simulink subsystem "Swerve_Drive_Module_sub"  (R2023b)
settings: Solver=VariableStepAuto  StartTime=0.0  StopTime=10.0  RelTol=1e-3
undefined symbols (not defined in the file): Drive_Motor_Control_Module_Angle_Error, Drive_Motor_Control_Scale_Factor, Drive_Motor_Control_Sign_Change_Deadband, Wheel_Speed_to_Motor_Speed
libraries: Controls_Components_lib x4, simulink x2
settings Model: Creator=ander  LastModifiedBy=ander

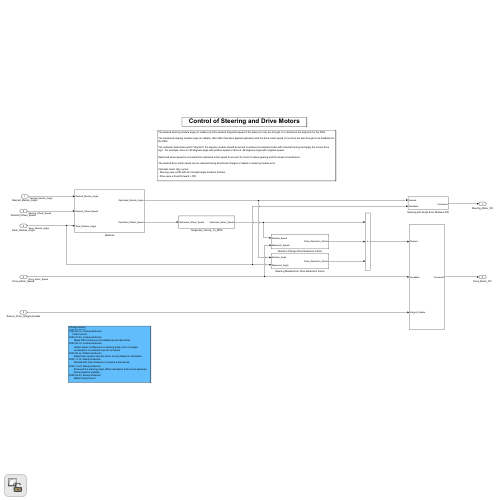
[thumbnail: Simulink's stored preview of the top-level diagram]
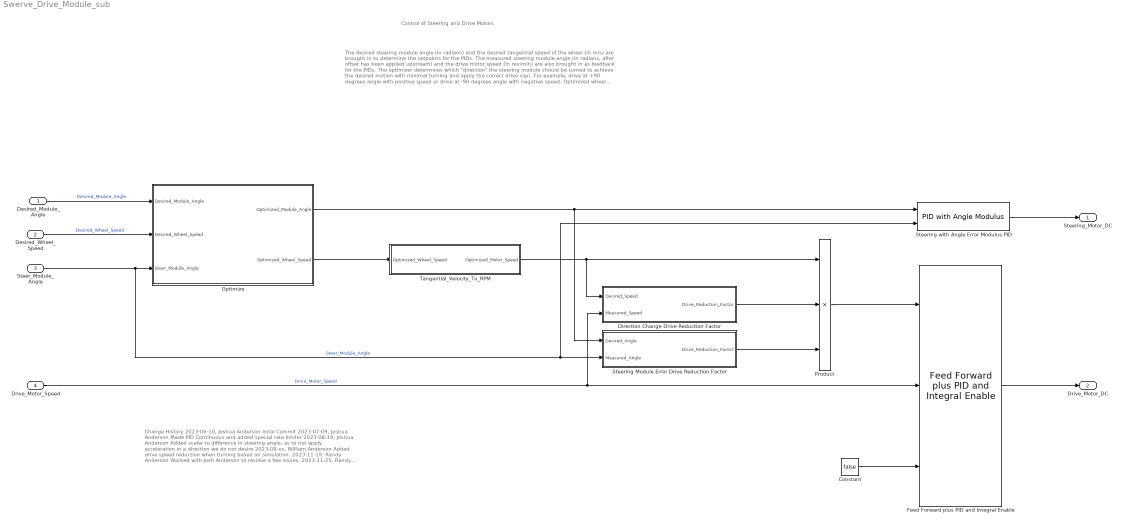
== system Swerve_Drive_Module_sub ==
  note: Change History
      | 2023-06-10, Joshua Anderson
      | Inital Commit
      | 2023-07-09, Joshua Anderson
      | Made PID Continuous and added special rate limiter
      | 2023-08-19, Joshua Anderson
      | Added scaler to difference in steering angle, as to not apply
      | acceleration in a direction we do not desire
      | 2023-08-xx, William Anderson
      | Added drive speed reduction when turning based on simulation.
      | 2023-11-19, Randy Anderson
      | Worked with Josh Anderson to resolve a few issues.
      | 2023-11-25, Randy Anderson
      | Removed the steering angle offset calculation and moved upstream.
      | Documentation updates.
      | 2025-03-05, Randy Anderson
      | Added integral enable
      | 2026-04-03, Randy Anderson
      | Removed integral enable (not used)
  note: Control of Steering and Drive Motors
  note: The desired steering module angle (in radians) and the desired tangential speed of the wheel (in m/s) are brought in to determine the setpoints for the PIDs.
      |
      | The measured steering module angle (in radians, after offset has been applied upstream) and the drive motor speed (in rev/min) are also brought in as feedback for the PIDs.
      |
      | The optimizer determines which "direction" the steering module should be turned to achieve the desired motion with minimal turning and apply the correct drive sign.  For example, drive at +90 degrees angle with positive speed or drive at -90 degrees angle with negative speed.
      |
      | Optimized wheel speed is converted into optimized motor speed to account for motor to wheel gearing and the wheel circumference.
      |
      | The desired drive motor speed can be reduced during directional changes or based on steering module error.
      |
      | Calculate motor duty cycles:
      | - Steering uses a PID with an included angle modulus function.
      | - Drive uses a Feed Forward + PID.
  Desired_Module_Angle : Inport  OutDataTypeStr=double  Unit=rad
  Desired_Wheel_Speed : Inport  Port=2  OutDataTypeStr=double  Unit=m/s
  Steer_Module_Angle : Inport  Port=3  OutDataTypeStr=double  Unit=rad
  Drive_Motor_Speed : Inport  Port=4  OutDataTypeStr=double  Unit=rpm
  Constant : Constant  Value=false
  Direction Change Drive Reduction Factor : Subsystem
  Feed Forward plus PID and Integral Enable : Controls_Components_lib/Feed Forward plus PID and Integral Enable  Gain_FF=Drive_Motor_Control_FF  Gain_P=Drive_Motor_Control_P  Gain_I=0  Gain_D=Drive_Motor_Control_D  FilterCoeff_D=Drive_Motor_Control_D_FilterCoeff  Limit_I_Upper=0  Limit_I_Lower=0  Limit_D_Upper=Drive_Motor_Control_D_UL  Limit_D_Lower=Drive_Motor_Control_D_LL  Limit_T_Upper=1  Limit_T_Lower=-1
  Optimize : Subsystem
  Product : Product  Inputs=3
  Steering Module Error Drive Reduction Factor : Subsystem
  Steering with Angle Error Modulus PID : Controls_Components_lib/PID with Angle Modulus  Gain_P=Steering_Motor_Control_P  Gain_I=Steering_Motor_Control_I  Gain_D=Steering_Motor_Control_D  FilterCoeff_D=Steering_Motor_Control_D_FilterCoeff  Limit_I_Upper=Steering_Motor_Control_I_UL  Limit_I_Lower=Steering_Motor_Control_I_LL  Limit_D_Upper=Steering_Motor_Control_D_UL  Limit_D_Lower=Steering_Motor_Control_D_LL  Limit_T_Upper=1  Limit_T_Lower=-1
  Tangential_Velocity_To_RPM : Subsystem
  Steering_Motor_DC : Outport  OutDataTypeStr=double  Unit=1
  Drive_Motor_DC : Outport  Port=2  OutDataTypeStr=double  Unit=1
  wires:
  Feed Forward plus PID and Integral Enable/1 -> Drive_Motor_DC/1
  Optimize/1(Optimized_Module_Angle) -> Steering with Angle Error Modulus PID/1, Steering Module Error Drive Reduction Factor/1(Desired_Angle)
  Steering with Angle Error Modulus PID/1 -> Steering_Motor_DC/1
  Steer_Module_Angle/1 -> Optimize/3(Steer_Module_Angle), Steering Module Error Drive Reduction Factor/2(Measured_Angle), Steering with Angle Error Modulus PID/2  "Steer_Module_Angle"
  Tangential_Velocity_To_RPM/1(Optimized_Motor_Speed) -> Product/1, Direction Change Drive Reduction Factor/1(Desired_Speed)
  Optimize/2(Optimized_Wheel_Speed) -> Tangential_Velocity_To_RPM/1(Optimized_Wheel_Speed)
  Desired_Wheel_Speed/1 -> Optimize/2(Desired_Wheel_Speed)  "Desired_Wheel_Speed"
  Desired_Module_Angle/1 -> Optimize/1(Desired_Module_Angle)  "Desired_Module_Angle"
  Drive_Motor_Speed/1 -> Direction Change Drive Reduction Factor/2(Measured_Speed), Feed Forward plus PID and Integral Enable/2  "Drive_Motor_Speed"
  Direction Change Drive Reduction Factor/1(Drive_Reduction_Factor) -> Product/2
  Product/1 -> Feed Forward plus PID and Integral Enable/1
  Steering Module Error Drive Reduction Factor/1(Drive_Reduction_Factor) -> Product/3
  Constant/1 -> Feed Forward plus PID and Integral Enable/3

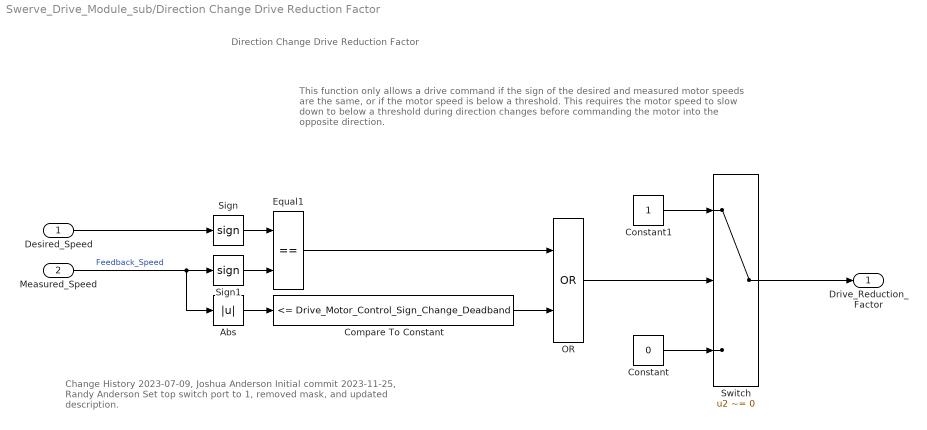
== system Swerve_Drive_Module_sub/Direction Change Drive Reduction Factor ==
  note: This function only allows a drive command if the sign of the desired and measured motor speeds are the same, or if the motor speed is below a threshold. This requires the motor speed to slow down to below a threshold during direction changes before commanding the motor into the opposite direction.
  note: Change History
      | 2023-07-09, Joshua Anderson
      | Initial commit
      | 2023-11-25, Randy Anderson
      | Set top switch port to 1, removed mask, and updated description.
  note: Direction Change Drive Reduction Factor
  Desired_Speed : Inport
  Measured_Speed : Inport  Port=2
  Abs : Abs  SaturateOnIntegerOverflow=off
  Compare To Constant : simulink/Logic and Bit Operations/Compare To Constant  relop=<=  const=Drive_Motor_Control_Sign_Change_Deadband  OutDataTypeStr=boolean
  Constant : Constant  Value=0
  Constant1 : Constant
  Equal1 : RelationalOperator  Operator===  OutDataTypeStr=boolean  RndMeth=Simplest  InputSameDT=off
  OR : Logic  Operator=OR  AllPortsSameDT=off  OutDataTypeStr=boolean
  Sign : Signum
  Sign1 : Signum
  Switch : Switch  Criteria=u2 ~= 0  SaturateOnIntegerOverflow=off  InputSameDT=off
  Drive_Reduction_Factor : Outport
  wires:
  Constant1/1 -> Switch/1
  OR/1 -> Switch/2
  Abs/1 -> Compare To Constant/1
  Measured_Speed/1 -> Abs/1, Sign1/1  "Feedback_Speed"
  Switch/1 -> Drive_Reduction_Factor/1
  Sign1/1 -> Equal1/2
  Desired_Speed/1 -> Sign/1
  Equal1/1 -> OR/1
  Constant/1 -> Switch/3
  Sign/1 -> Equal1/1
  Compare To Constant/1 -> OR/2

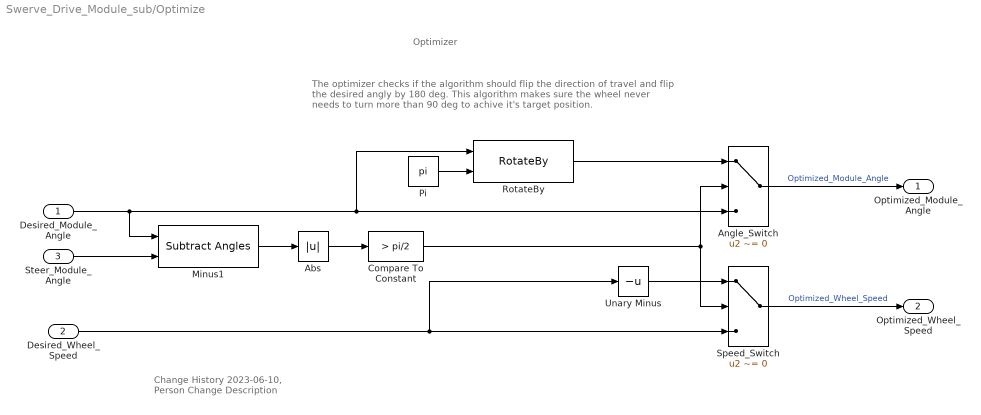
== system Swerve_Drive_Module_sub/Optimize ==
  note: Optimizer
  note: Change History
      | 2023-06-10, Person
      | Change Description
  note: The optimizer checks if the algorithm should flip the direction of travel and flip the desired angly by 180 deg. This algorithm makes sure the wheel never needs to turn more than 90 deg to achive it's target position.
  Desired_Module_Angle : Inport  OutDataTypeStr=double  Unit=rad
  Desired_Wheel_Speed : Inport  Port=2  OutDataTypeStr=double  Unit=m/s
  Steer_Module_Angle : Inport  Port=3  OutDataTypeStr=double  Unit=rad
  Abs : Abs  SaturateOnIntegerOverflow=off
  Angle_Switch : Switch  Criteria=u2 ~= 0  SaturateOnIntegerOverflow=off  InputSameDT=off
  Compare To Constant : simulink/Logic and Bit Operations/Compare To Constant  relop=>  const=pi/2  OutDataTypeStr=boolean
  Minus1 : Controls_Components_lib/Subtract Angles  SystemSampleTime=-1  VariantActivationTime=update diagram  AllowFlexibleInterface=on  Latency=0  AutoFrameSizeCalculation=off
  Pi : Constant  Value=pi  OutDataTypeStr=Inherit: Inherit via back propagation
  RotateBy : Controls_Components_lib/RotateBy  SystemSampleTime=-1  VariantActivationTime=update diagram  AllowFlexibleInterface=on  Latency=0  AutoFrameSizeCalculation=off
  Speed_Switch : Switch  Criteria=u2 ~= 0  SaturateOnIntegerOverflow=off  InputSameDT=off
  Unary Minus : UnaryMinus
  Optimized_Module_Angle : Outport  OutDataTypeStr=double  Unit=rad
  Optimized_Wheel_Speed : Outport  Port=2  OutDataTypeStr=double  Unit=m/s
  wires:
  RotateBy/1 -> Angle_Switch/1
  Speed_Switch/1 -> Optimized_Wheel_Speed/1  "Optimized_Wheel_Speed"
  Angle_Switch/1 -> Optimized_Module_Angle/1  "Optimized_Module_Angle"
  Pi/1 -> RotateBy/2
  Unary Minus/1 -> Speed_Switch/1
  Compare To Constant/1 -> Speed_Switch/2, Angle_Switch/2
  Desired_Wheel_Speed/1 -> Speed_Switch/3, Unary Minus/1
  Abs/1 -> Compare To Constant/1
  Minus1/1 -> Abs/1
  Steer_Module_Angle/1 -> Minus1/2
  Desired_Module_Angle/1 -> Angle_Switch/3, RotateBy/1, Minus1/1

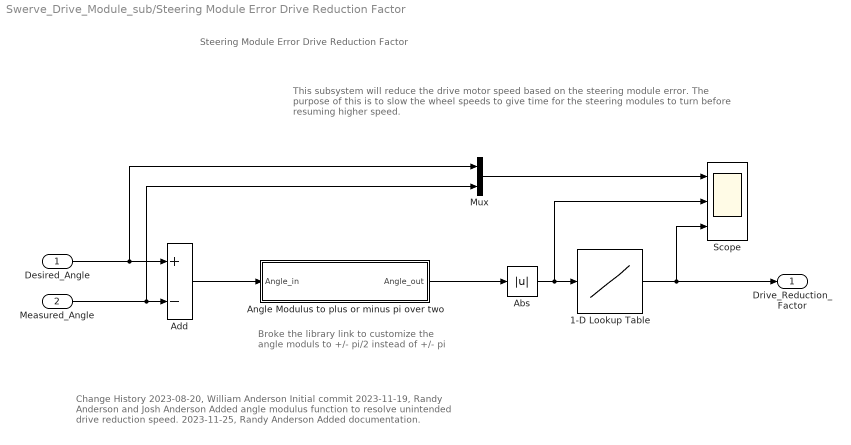
== system Swerve_Drive_Module_sub/Steering Module Error Drive Reduction Factor ==
  note: Change History
      | 2023-08-20, William Anderson
      | Initial commit
      | 2023-11-19, Randy Anderson and Josh Anderson
      | Added angle modulus function to resolve unintended drive reduction speed.
      | 2023-11-25, Randy Anderson
      | Added documentation.
  note: Steering Module Error Drive Reduction Factor
  note: This subsystem will reduce the drive motor speed based on the steering module error. The purpose of this is to slow the wheel speeds to give time for the steering modules to turn before resuming higher speed.
  note: Broke the library link to customize the
      | angle moduls to +/- pi/2 instead of +/- pi
  Desired_Angle : Inport
  Measured_Angle : Inport  Port=2
  1-D Lookup Table : Lookup_n-D  NumberOfTableDimensions=1  BreakpointsForDimension1=Drive_Motor_Control_Module_Angle_Error  Table=Drive_Motor_Control_Scale_Factor  ExtrapMethod=Clip  InternalRulePriority=Speed  RndMeth=Simplest
  Abs : Abs  SaturateOnIntegerOverflow=off
  Add : Sum  Inputs=+-
  Angle Modulus to plus or minus pi over two : Subsystem
  Mux : Mux  Inputs=2
  Scope : Scope  NumInputPorts=3
  Drive_Reduction_Factor : Outport
  wires:
  Add/1 -> Angle Modulus to plus or minus pi over two/1(Angle_in)
  Angle Modulus to plus or minus pi over two/1(Angle_out) -> Abs/1
  Desired_Angle/1 -> Mux/1, Add/1
  Measured_Angle/1 -> Mux/2, Add/2
  Abs/1 -> Scope/2, 1-D Lookup Table/1
  1-D Lookup Table/1 -> Scope/3, Drive_Reduction_Factor/1
  Mux/1 -> Scope/1

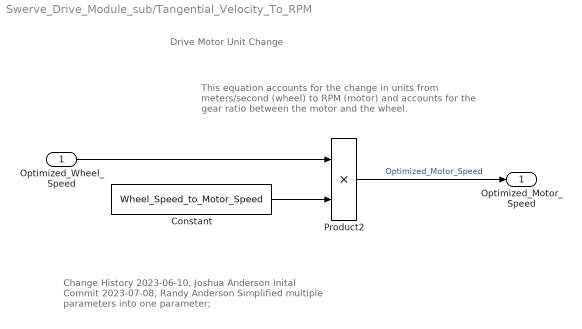
== system Swerve_Drive_Module_sub/Tangential_Velocity_To_RPM ==
  note: Drive Motor Unit Change
  note: Change History
      | 2023-06-10, Joshua Anderson
      | Inital Commit
      | 2023-07-08, Randy Anderson
      | Simplified multiple parameters into one parameter;
  note: This equation accounts for the change in units from meters/second (wheel) to RPM (motor) and accounts for the gear ratio between the motor and the wheel.
  Optimized_Wheel_Speed : Inport  Unit=m/s
  Constant : Constant  Value=Wheel_Speed_to_Motor_Speed
  Product2 : Product
  Optimized_Motor_Speed : Outport  Unit=rpm
  wires:
  Constant/1 -> Product2/2
  Optimized_Wheel_Speed/1 -> Product2/1
  Product2/1 -> Optimized_Motor_Speed/1  "Optimized_Motor_Speed"

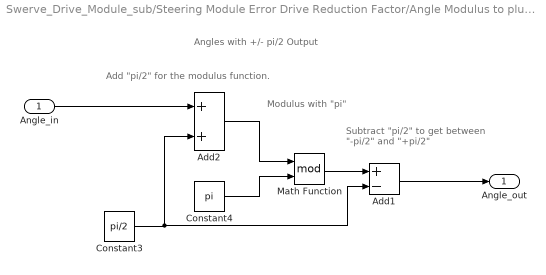
== system Swerve_Drive_Module_sub/Steering Module Error Drive Reduction Factor/Angle Modulus to plus or minus pi over two ==
  note: Add "pi/2" for the modulus function.
  note: Modulus with "pi"
  note: Subtract "pi/2" to get
      | between "-pi/2" and "+pi/2"
  note: Angles with +/- pi/2 Output
  Angle_in : Inport
  Add1 : Sum  Inputs=+-
  Add2 : Sum
  Constant3 : Constant  Value=pi/2
  Constant4 : Constant  Value=pi
  Math Function : Math  Operator=mod
  Angle_out : Outport
  wires:
  Angle_in/1 -> Add2/1
  Constant3/1 -> Add1/2, Add2/2
  Add2/1 -> Math Function/1
  Constant4/1 -> Math Function/2
  Math Function/1 -> Add1/1
  Add1/1 -> Angle_out/1
